simulink model "palombaro"  (R2026b)
settings: Solver=ode45  StopTime=Tfine  MaxStep=0.005
PreLoadFcn:
  | addpath(fileparts(which('palombaro'))); run('parametri_gemello.m');
values from neighbouring files (symbols this model uses):
  c_ = 0.0044    [parametri_gemello.m]
  dp_max = 2000    [parametri_gemello.m]
  dp_onoff = 700    [esporta_gemello_f4.m]    (also in parametri_gemello.m = 300; progetto_controllori.m; soglia_gioco.m; tracking_5_4.m)
  g_ = 9.806    [parametri_gemello.m]
  h0_ = 0    [confronto_f4.m]    (also in esporta_gemello_f4.m; parametri_gemello.m; progetto_controllori.m; soglia_gioco.m)
  H_bolla = 0.20    (= 0.2)    [parametri_gemello.m]
  isteresi = 0.005    [parametri_gemello.m]    (also in soglia_gioco.m; tracking_5_4.m)
  Kd_h = 40000    [controllori.mat]    (also in parametri_gemello.m = 29000; progetto_controllori.m = guadagni(2); soglia_gioco.m = 0; tracking_5_4.m = g.Kd_h)
  Ki_h = 1187.5    [controllori.mat]    (also in parametri_gemello.m = 0; progetto_controllori.m = guadagni(3); soglia_gioco.m = 0; tracking_5_4.m = g.Ki_h)
  Ki_p = 0.4    [controllori.mat]    (also in esporta_gemello_f4.m = g.Ki_p; parametri_gemello.m; soglia_gioco.m = taratura{j, 2}; tracking_5_4.m)
  Kp_h = 47500    [controllori.mat]    (also in parametri_gemello.m = 47000; progetto_controllori.m = guadagni(1); soglia_gioco.m = 1; tracking_5_4.m = g.Kp_h)
  Kp_p = 0.02    [confronto_f4.m]    (also in controllori.mat; esporta_gemello_f4.m = g.Kp_p; parametri_gemello.m; soglia_gioco.m)
  Ks = 0.16    [parametri_gemello.m]
  m_ = 997.6*(Vs_ + Vb_)    (= 0.00309256)    [parametri_gemello.m]
  meff_ = m_*1.5    (= 0.00463884)    [parametri_gemello.m]
  modo_controllo = 1    [confronto_f4.m]    (also in esporta_gemello_f4.m; parametri_gemello.m = 0; progetto_controllori.m; soglia_gioco.m)
  modo_esterno = 1    [parametri_gemello.m]    (also in soglia_gioco.m; tracking_5_4.m)
  modo_pressione = 0    [confronto_f4.m]    (also in esporta_gemello_f4.m; parametri_gemello.m; soglia_gioco.m; tracking_5_4.m)
  N_h = g.N_h    [confronto_f4.m]    (also in controllori.mat = 10; esporta_gemello_f4.m; parametri_gemello.m = 10; soglia_gioco.m)
  p0_ff = p0_    [esporta_gemello_f4.m]    (also in parametri_gemello.m = 101544; progetto_controllori.m = p0_ + errore_p0; soglia_gioco.m = p0_ + 500; tracking_5_4.m)
  p_atm = p0_ + 1500    [confronto_f4.m]    (also in esporta_gemello_f4.m = 101640; parametri_gemello.m = 101640; progetto_controllori.m = 101640; soglia_gioco.m)
  pb_ = p0_ + rho_g*H_bolla    (= 103500.49312)    [parametri_gemello.m]
  rho_g = 997.6*9.806    (= 9782.4656)    [parametri_gemello.m]
  ritardo_camera = 0.156    [parametri_gemello.m]
  rumore_h = 0.32e-3    (= 0.00032)    [parametri_gemello.m]
  rumore_on = 1    [confronto_f4.m]    (also in esporta_gemello_f4.m; parametri_gemello.m; progetto_controllori.m; soglia_gioco.m)
  rumore_p = 2.5    [parametri_gemello.m]
  T_camera = 1/60    (= 0.0166666666667)    [parametri_gemello.m]
  T_pressione = 0.01    [parametri_gemello.m]
  tau_perdita = 90*60    (= 5400)    [parametri_gemello.m]
  Ts_h = 0.03    [controllori.mat]    (also in parametri_gemello.m)
  Ts_p = 0.01    [controllori.mat]    (also in parametri_gemello.m)
  u0_ctrl = 90    [confronto_f4.m]    (also in esporta_gemello_f4.m = 66; parametri_gemello.m = 36; progetto_controllori.m = 66; soglia_gioco.m)
  u_chiusura = 116    [confronto_f4.m]    (also in esporta_gemello_f4.m = 66; parametri_gemello.m = 36; progetto_controllori.m = 66; soglia_gioco.m)
  Vb_ = 2.1e-6    (= 2.1e-06)    [parametri_gemello.m]
  Veff = 640    [parametri_gemello.m]
  vel_servo = 200    [parametri_gemello.m]
  Vs_ = 1.0e-6    (= 1e-06)    [parametri_gemello.m]
libraries: slpidlib x2
settings Model: Creator=gabrielecaruso  LastModifiedBy=gabrielecaruso

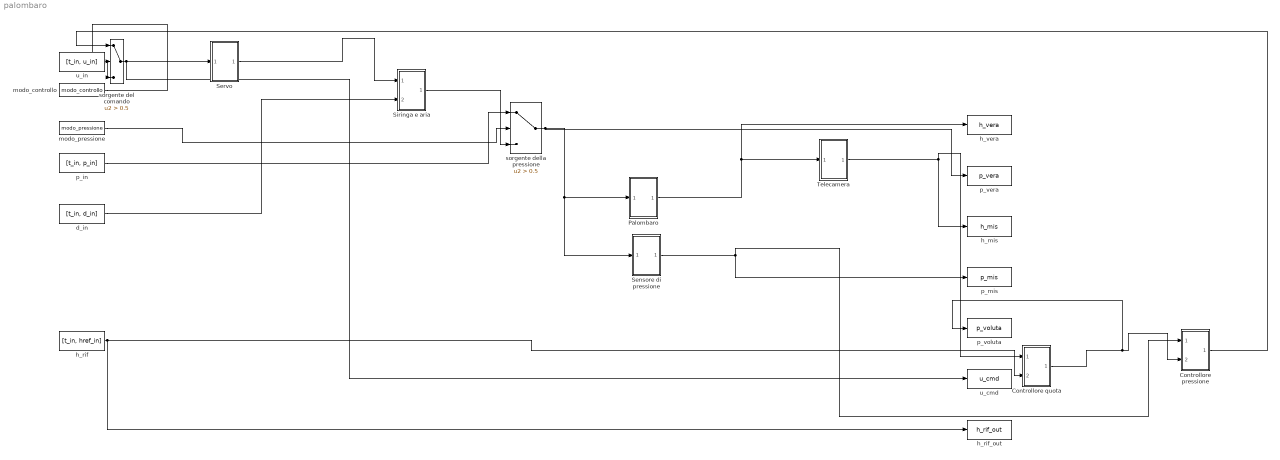
== system palombaro ==
  Controllore pressione : Subsystem
  Controllore quota : Subsystem
  Palombaro : Subsystem
  Sensore di pressione : Subsystem
  Servo : Subsystem
  Siringa e aria : Subsystem
  Telecamera : Subsystem
  d_in : FromWorkspace  VariableName=[t_in, d_in]  OutputAfterFinalValue=Holding final value
  h_mis : ToWorkspace  VariableName=h_mis  SaveFormat=Timeseries  SampleTime=-1
  h_rif : FromWorkspace  VariableName=[t_in, href_in]  OutputAfterFinalValue=Holding final value
  h_rif_out : ToWorkspace  VariableName=h_rif_out  SaveFormat=Timeseries  SampleTime=-1
  h_vera : ToWorkspace  VariableName=h_vera  SaveFormat=Timeseries  SampleTime=-1
  modo_controllo : Constant  Value=modo_controllo
  modo_pressione : Constant  Value=modo_pressione
  p_in : FromWorkspace  VariableName=[t_in, p_in]  OutputAfterFinalValue=Holding final value
  p_mis : ToWorkspace  VariableName=p_mis  SaveFormat=Timeseries  SampleTime=-1
  p_vera : ToWorkspace  VariableName=p_vera  SaveFormat=Timeseries  SampleTime=-1
  p_voluta : ToWorkspace  VariableName=p_voluta  SaveFormat=Timeseries  SampleTime=-1
  sorgente del comando : Switch  Criteria=u2 > Threshold  Threshold=0.5  SaturateOnIntegerOverflow=off  InputSameDT=off
  sorgente della pressione : Switch  Criteria=u2 > Threshold  Threshold=0.5  SaturateOnIntegerOverflow=off  InputSameDT=off
  u_cmd : ToWorkspace  VariableName=u_cmd  SaveFormat=Timeseries  SampleTime=-1
  u_in : FromWorkspace  VariableName=[t_in, u_in]  Interpolate=off  OutputAfterFinalValue=Holding final value
  wires:
  u_in/1 -> sorgente del comando/3
  modo_controllo/1 -> sorgente del comando/2
  sorgente del comando/1 -> Servo/1(In1), u_cmd/1
  p_in/1 -> sorgente della pressione/1
  modo_pressione/1 -> sorgente della pressione/2
  sorgente della pressione/1 -> Sensore di pressione/1(In1), Palombaro/1(In1), p_vera/1
  h_rif/1 -> Controllore quota/2(In2), h_rif_out/1
  Servo/1(Out1) -> Siringa e aria/1(In1)
  d_in/1 -> Siringa e aria/2(In2)
  Siringa e aria/1(Out1) -> sorgente della pressione/3
  Controllore quota/1(Out1) -> Controllore pressione/2(In2), p_voluta/1
  Controllore pressione/1(Out1) -> sorgente del comando/1
  Palombaro/1(Out1) -> h_vera/1, Telecamera/1(In1)
  Sensore di pressione/1(Out1) -> Controllore pressione/1(In1), p_mis/1
  Telecamera/1(Out1) -> Controllore quota/1(In1), h_mis/1

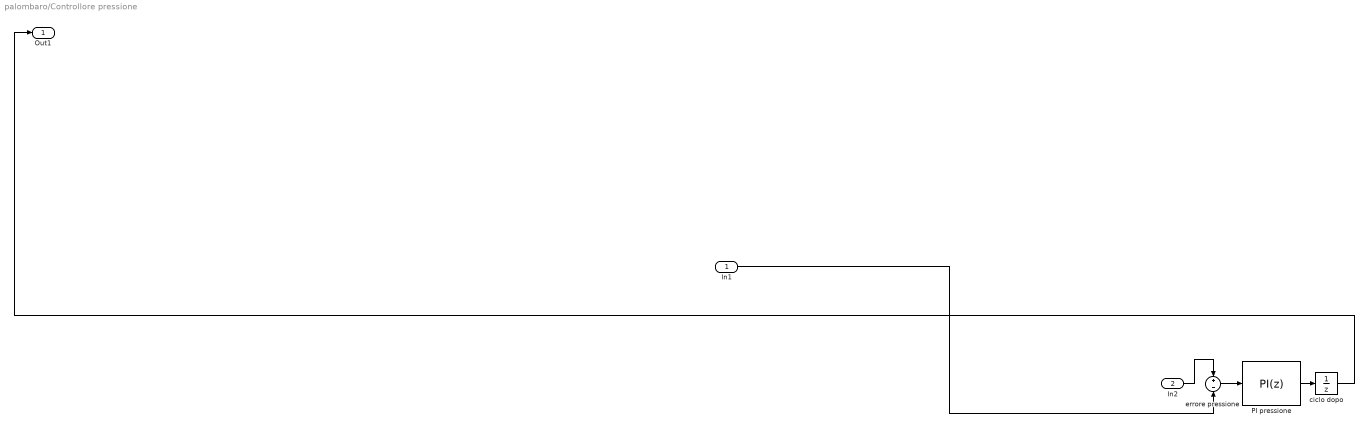
== system palombaro/Controllore pressione ==
  In1 : Inport
  In2 : Inport  Port=2
  PI pressione : slpidlib/PID Controller  Controller=PI  Form=Parallel  TimeDomain=Discrete-time  UseExternalTs=off  SampleTime=Ts_p  IntegratorMethod=Forward Euler  FilterMethod=Forward Euler  ControllerParametersSource=internal  P=Kp_p  I=Ki_p  UseKiTs=off  D=0  UseExternalDerivativeSource=off  N=100  UseFilter=on  TunerSelectOption=Transfer Function Based (PID Tuner App)  InitialConditionSource=internal  InitialConditionForIntegrator=u0_ctrl  InitialConditionForFilter=0  DifferentiatorICPrevScaledInput=0  ExternalReset=none  TrackingMode=off  Kt=1  LimitOutput=on  SatLimitsSource=internal  UpperSaturationLimit=146  LowerSaturationLimit=36  LinearizeAsGain=off  AntiWindupMode=clamping  Kb=1  LimitIntegrator=off  UpperIntegratorSaturationLimit=inf  LowerIntegratorSaturationLimit=-inf  POutMin=[]  POutMax=[]  IOutMin=[]  IOutMax=[]  DOutMin=[]  DOutMax=[]  NOutMin=[]  NOutMax=[]  SumOutMin=[]  SumOutMax=[]  SaturationOutMin=[]  SaturationOutMax=[]  PParamMin=[]  PParamMax=[]  IParamMin=[]  IParamMax=[]  DParamMin=[]  DParamMax=[]  NParamMin=[]  NParamMax=[]  KbParamMin=[]  KbParamMax=[]  KtParamMin=[]  KtParamMax=[]  KbOutMin=[]  KbOutMax=[]  KtOutMin=[]  KtOutMax=[]  IntegratorOutMin=[]  IntegratorOutMax=[]  FilterOutMin=[]  FilterOutMax=[]  SumI1OutMin=[]  SumI1OutMax=[]  SumI2OutMin=[]  SumI2OutMax=[]  SumI3OutMin=[]  SumI3OutMax=[]  SumI4OutMin=[]  SumI4OutMax=[]  SumDOutMin=[]  SumDOutMax=[]  DifferentiatorOutMin=[]  DifferentiatorOutMax=[]  FilterDiffOutCoefMin=[]  FilterDiffOutCoefMax=[]  ReciprocalOutMin=[]  ReciprocalOutMax=[]  SumDenOutMin=[]  SumDenOutMax=[]  SumNumOutMin=[]  SumNumOutMax=[]  DivideOutMin=[]  DivideOutMax=[]  UdiffTsProdOutMin=[]  UdiffTsProdOutMax=[]  NTsProdOutMin=[]  NTsProdOutMax=[]  UintegralTsProdOutMin=[]  UintegralTsProdOutMax=[]  UngainTsProdOutMin=[]  UngainTsProdOutMax=[]  ClampingZeroOutDataTypeStr=Inherit: Inherit via back propagation  ClampingZeroOutMin=[]  ClampingZeroOutMax=[]  FilterDenConstantOutDataTypeStr=Inherit: Inherit via back propagation  FilterDenConstantOutMin=[]  FilterDenConstantOutMax=[]  PCopyOutDataTypeStr=Inherit: Inherit via back propagation  PCopyOutMin=[]  PCopyOutMax=[]  NCopyOutDataTypeStr=Inherit: Inherit via back propagation  NCopyOutMin=[]  NCopyOutMax=[]  IntegratorContinuousStateAttributes=''  IntegratorStateMustResolveToSignalObject=off  IntegratorRTWStateStorageClass=Auto  FilterContinuousStateAttributes=''  FilterStateMustResolveToSignalObject=off  FilterRTWStateStorageClass=Auto  ParallelPVariant=InternalParameters  IdealPVariant=Disabled  IVariant=InternalParameters  DVariant=Disabled  IntegratorVariant=Discrete  SatVariant=Enabled  AWVariant=DiscClampingParallel  PCopyVariant=Disabled  TRVariant=Disabled  FdbkBlocksVariant=Forward  IdealPFdbkVariant=Disabled  SatFdbkVariant=Disabled  DerivativeFilterVariant=Disabled  NVariant=Disabled  NCopyVariant=Disabled_SignalSpec  FilterICVariant=Disabled  IntegratorICVariant=InternalICs  ExternalResetVariant=Disabled  TRSumVariant=Passthrough  SumFdbkVariant=Disabled  SumVariant=Sum_PI  TsampFilterVariant=InternalTs  TsampNgainVariant=Passthrough  TsampIntegralVariant=Disabled_SignalSpec  ExternalSaturationOutDataTypeStr=Inherit: Same as second input  DerivativeSourceVariant=Disabled  PreIntVariant=InternalPreInt
      settings: LibrarySourceBlock=simulink/Discrete/Discrete PID Controller
  ciclo dopo : UnitDelay  InitialCondition=u0_ctrl  SampleTime=Ts_p
  errore pressione : Sum  Inputs=+-
  Out1 : Outport
  wires:
  ciclo dopo/1 -> Out1/1
  PI pressione/1 -> ciclo dopo/1
  In1/1 -> errore pressione/2
  In2/1 -> errore pressione/1
  errore pressione/1 -> PI pressione/1

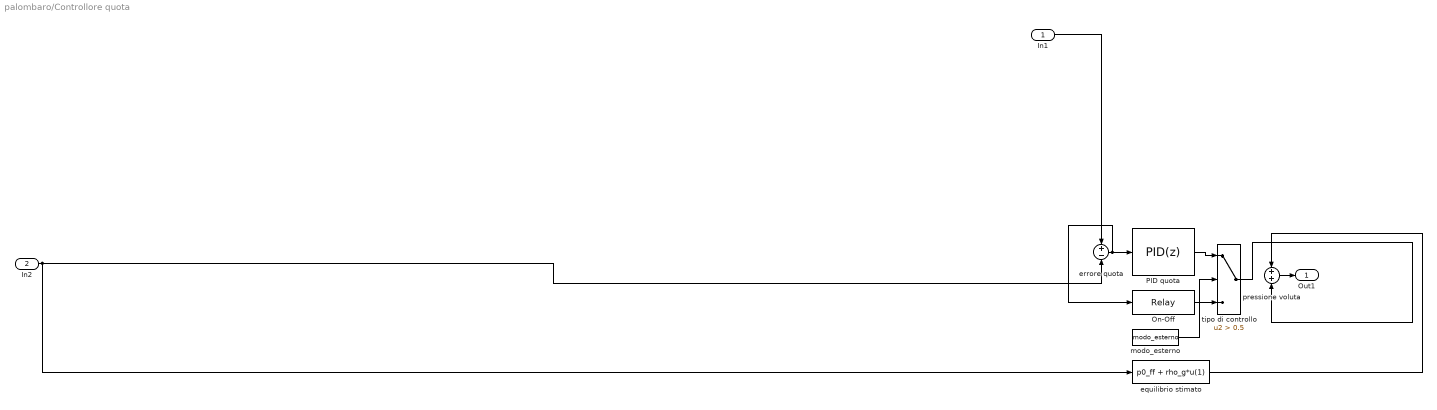
== system palombaro/Controllore quota ==
  In1 : Inport
  In2 : Inport  Port=2
  On-Off : Relay  OnSwitchValue=isteresi  OffSwitchValue=-isteresi  OnOutputValue=dp_onoff  OffOutputValue=-dp_onoff
  PID quota : slpidlib/PID Controller  Controller=PID  Form=Parallel  TimeDomain=Discrete-time  UseExternalTs=off  SampleTime=Ts_h  IntegratorMethod=Forward Euler  FilterMethod=Forward Euler  ControllerParametersSource=internal  P=Kp_h  I=Ki_h  UseKiTs=off  D=Kd_h  UseExternalDerivativeSource=off  N=N_h  UseFilter=on  TunerSelectOption=Transfer Function Based (PID Tuner App)  InitialConditionSource=internal  InitialConditionForIntegrator=0  InitialConditionForFilter=0  DifferentiatorICPrevScaledInput=0  ExternalReset=none  TrackingMode=off  Kt=1  LimitOutput=on  SatLimitsSource=internal  UpperSaturationLimit=dp_max  LowerSaturationLimit=-dp_max  LinearizeAsGain=off  AntiWindupMode=clamping  Kb=1  LimitIntegrator=off  UpperIntegratorSaturationLimit=inf  LowerIntegratorSaturationLimit=-inf  POutMin=[]  POutMax=[]  IOutMin=[]  IOutMax=[]  DOutMin=[]  DOutMax=[]  NOutMin=[]  NOutMax=[]  SumOutMin=[]  SumOutMax=[]  SaturationOutMin=[]  SaturationOutMax=[]  PParamMin=[]  PParamMax=[]  IParamMin=[]  IParamMax=[]  DParamMin=[]  DParamMax=[]  NParamMin=[]  NParamMax=[]  KbParamMin=[]  KbParamMax=[]  KtParamMin=[]  KtParamMax=[]  KbOutMin=[]  KbOutMax=[]  KtOutMin=[]  KtOutMax=[]  IntegratorOutMin=[]  IntegratorOutMax=[]  FilterOutMin=[]  FilterOutMax=[]  SumI1OutMin=[]  SumI1OutMax=[]  SumI2OutMin=[]  SumI2OutMax=[]  SumI3OutMin=[]  SumI3OutMax=[]  SumI4OutMin=[]  SumI4OutMax=[]  SumDOutMin=[]  SumDOutMax=[]  DifferentiatorOutMin=[]  DifferentiatorOutMax=[]  FilterDiffOutCoefMin=[]  FilterDiffOutCoefMax=[]  ReciprocalOutMin=[]  ReciprocalOutMax=[]  SumDenOutMin=[]  SumDenOutMax=[]  SumNumOutMin=[]  SumNumOutMax=[]  DivideOutMin=[]  DivideOutMax=[]  UdiffTsProdOutMin=[]  UdiffTsProdOutMax=[]  NTsProdOutMin=[]  NTsProdOutMax=[]  UintegralTsProdOutMin=[]  UintegralTsProdOutMax=[]  UngainTsProdOutMin=[]  UngainTsProdOutMax=[]  ClampingZeroOutDataTypeStr=Inherit: Inherit via back propagation  ClampingZeroOutMin=[]  ClampingZeroOutMax=[]  FilterDenConstantOutDataTypeStr=Inherit: Inherit via back propagation  FilterDenConstantOutMin=[]  FilterDenConstantOutMax=[]  PCopyOutDataTypeStr=Inherit: Inherit via back propagation  PCopyOutMin=[]  PCopyOutMax=[]  NCopyOutDataTypeStr=Inherit: Inherit via back propagation  NCopyOutMin=[]  NCopyOutMax=[]  IntegratorContinuousStateAttributes=''  IntegratorStateMustResolveToSignalObject=off  IntegratorRTWStateStorageClass=Auto  FilterContinuousStateAttributes=''  FilterStateMustResolveToSignalObject=off  FilterRTWStateStorageClass=Auto  ParallelPVariant=InternalParameters  IdealPVariant=Disabled  IVariant=InternalParameters  DVariant=InternalParameters  IntegratorVariant=Discrete  SatVariant=Enabled  AWVariant=DiscClampingParallel  PCopyVariant=Disabled  TRVariant=Disabled  FdbkBlocksVariant=Forward  IdealPFdbkVariant=Disabled  SatFdbkVariant=Disabled  DerivativeFilterVariant=ForwardEulerFilter  NVariant=InternalParameters  NCopyVariant=Disabled  FilterICVariant=InternalICsFilter  IntegratorICVariant=InternalICs  ExternalResetVariant=Disabled  TRSumVariant=Passthrough  SumFdbkVariant=Disabled  SumVariant=Sum_PID  TsampFilterVariant=InternalTs  TsampNgainVariant=Passthrough  TsampIntegralVariant=Disabled_SignalSpec  ExternalSaturationOutDataTypeStr=Inherit: Same as second input  DerivativeSourceVariant=ErrorSignal  PreIntVariant=InternalPreInt
      settings: LibrarySourceBlock=simulink/Discrete/Discrete PID Controller
  equilibrio stimato : Fcn  Expr=p0_ff + rho_g*u(1)
  errore quota : Sum  Inputs=+-
  modo_esterno : Constant  Value=modo_esterno
  pressione voluta : Sum
  tipo di controllo : Switch  Criteria=u2 > Threshold  Threshold=0.5  SaturateOnIntegerOverflow=off  InputSameDT=off
  Out1 : Outport
  wires:
  In2/1 -> equilibrio stimato/1, errore quota/2
  pressione voluta/1 -> Out1/1
  In1/1 -> errore quota/1
  modo_esterno/1 -> tipo di controllo/2
  tipo di controllo/1 -> pressione voluta/2
  equilibrio stimato/1 -> pressione voluta/1
  On-Off/1 -> tipo di controllo/3
  errore quota/1 -> PID quota/1, On-Off/1
  PID quota/1 -> tipo di controllo/1

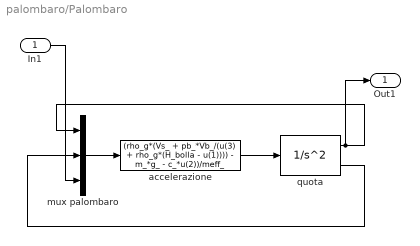
== system palombaro/Palombaro ==
  In1 : Inport
  accelerazione : Fcn  Expr=(rho_g*(Vs_ + pb_*Vb_/(u(3) + rho_g*(H_bolla - u(1)))) - m_*g_ - c_*u(2))/meff_
  mux palombaro : Mux  Inputs=3
  quota : SecondOrderIntegrator  ICX=h0_  LimitX=on  UpperLimitX=H_cima  LowerLimitX=0  ICDXDT=v0_  LimitDXDT=on
  Out1 : Outport
  wires:
  In1/1 -> mux palombaro/3
  accelerazione/1 -> quota/1
  quota/2 -> mux palombaro/2
  mux palombaro/1 -> accelerazione/1
  quota/1 -> Out1/1, mux palombaro/1

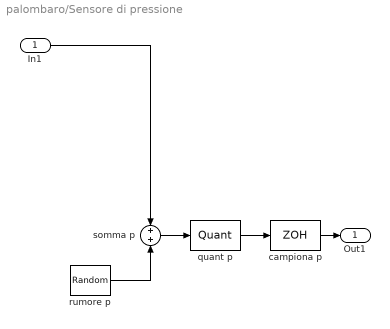
== system palombaro/Sensore di pressione ==
  In1 : Inport
  campiona p : ZeroOrderHold  SampleTime=T_pressione
  quant p : Quantizer  QuantizationInterval=quant_p
  rumore p : RandomNumber  Variance=(rumore_on*rumore_p)^2  Seed=11  SampleTime=T_pressione
  somma p : Sum
  Out1 : Outport
  wires:
  campiona p/1 -> Out1/1
  quant p/1 -> campiona p/1
  In1/1 -> somma p/1
  rumore p/1 -> somma p/2
  somma p/1 -> quant p/1

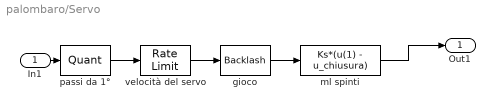
== system palombaro/Servo ==
  In1 : Inport
  gioco : Backlash  BacklashWidth=gioco_servo  InitialOutput=u_chiusura
  ml spinti : Fcn  Expr=Ks*(u(1) - u_chiusura)
  passi da 1° : Quantizer  QuantizationInterval=passo_servo
  velocità del servo : RateLimiter  RisingSlewLimit=vel_servo  FallingSlewLimit=-vel_servo  SampleTimeMode=inherited  InitialCondition=u_chiusura
  Out1 : Outport
  wires:
  ml spinti/1 -> Out1/1
  In1/1 -> passi da 1°/1
  gioco/1 -> ml spinti/1
  velocità del servo/1 -> gioco/1
  passi da 1°/1 -> velocità del servo/1

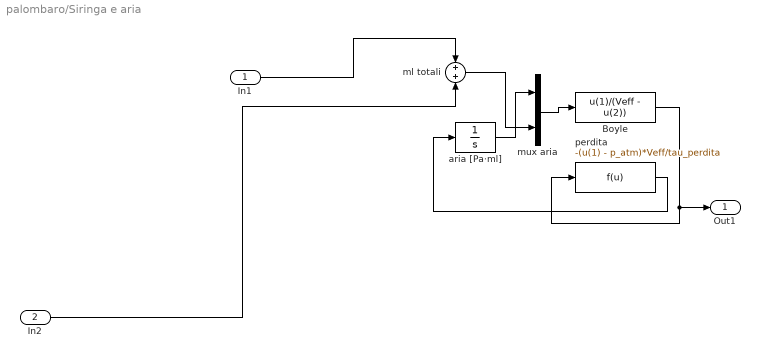
== system palombaro/Siringa e aria ==
  In1 : Inport
  In2 : Inport  Port=2
  Boyle : Fcn  Expr=u(1)/(Veff - u(2))
  aria [Pa·ml] : Integrator  InitialCondition=p_atm*Veff
  ml totali : Sum
  mux aria : Mux  Inputs=2
  perdita : Fcn  Expr=-(u(1) - p_atm)*Veff/tau_perdita
  Out1 : Outport
  wires:
  In1/1 -> ml totali/1
  In2/1 -> ml totali/2
  perdita/1 -> aria [Pa·ml]/1
  Boyle/1 -> Out1/1, perdita/1
  mux aria/1 -> Boyle/1
  aria [Pa·ml]/1 -> mux aria/1
  ml totali/1 -> mux aria/2

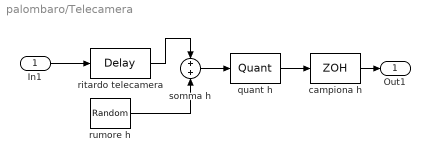
== system palombaro/Telecamera ==
  In1 : Inport
  campiona h : ZeroOrderHold  SampleTime=T_camera
  quant h : Quantizer  QuantizationInterval=quant_h
  ritardo telecamera : TransportDelay  DelayTime=ritardo_camera  InitialOutput=h0_
  rumore h : RandomNumber  Variance=(rumore_on*rumore_h)^2  Seed=23  SampleTime=T_camera
  somma h : Sum
  Out1 : Outport
  wires:
  In1/1 -> ritardo telecamera/1
  rumore h/1 -> somma h/2
  campiona h/1 -> Out1/1
  quant h/1 -> campiona h/1
  somma h/1 -> quant h/1
  ritardo telecamera/1 -> somma h/1
